simulink model "SimplePropellerModel"  (R2025b)
settings: Solver=VariableStepAuto  StartTime=0.0  StopTime=20  RelTol=1e-3
undefined symbols (not defined in the file): km, kT, spinDir
libraries: simulink x1
settings Model: Creator=esmithzb  LastModifiedBy=David
settings DebuggingCC: UnderspecifiedInitializationDetection=Classic  MergeDetectMultiDrivingBlocksExec=none
settings ModelReferenceCC: PropagateSignalLabelsOutOfModel=off

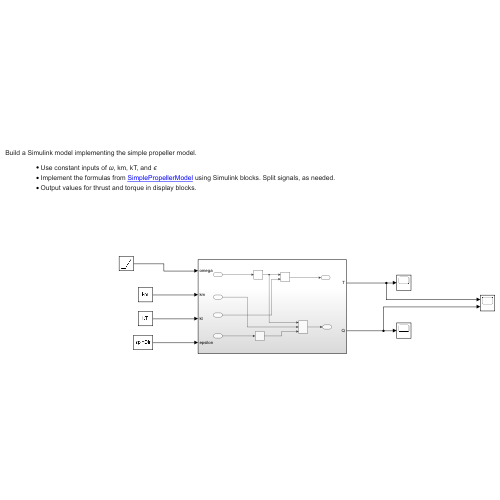
[thumbnail: Simulink's stored preview of the top-level diagram]
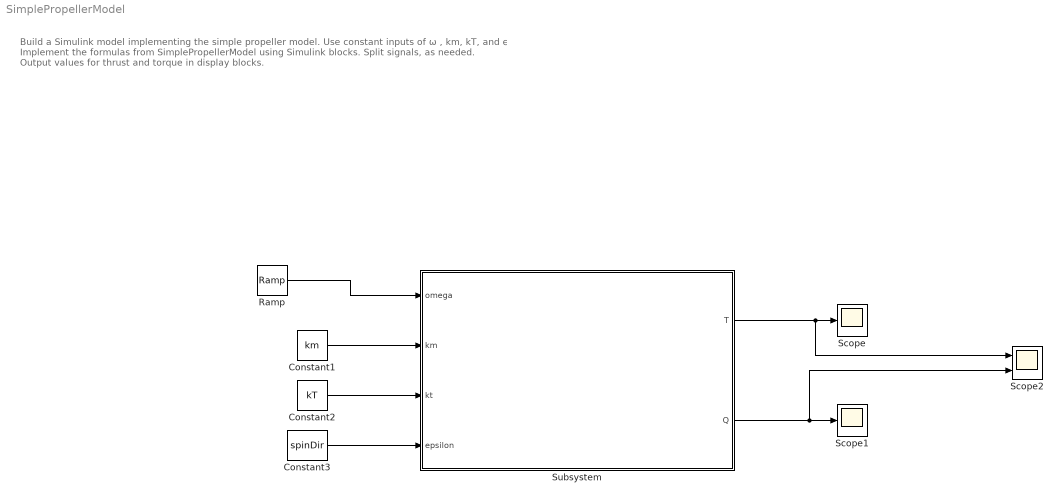
== system SimplePropellerModel ==
  note: Build a Simulink model implementing the simple propeller model.
      | Use constant inputs of ω , km, kT, and ϵ
      | Implement the formulas from SimplePropellerModel using Simulink blocks. Split signals, as needed.
      | Output values for thrust and torque in display blocks.
  Constant1 : Constant  Value=km
  Constant2 : Constant  Value=kT
  Constant3 : Constant  Value=spinDir
  Ramp : simulink/Sources/Ramp  slope=4.5  start=0  InitialOutput=0
  Scope : Scope
      settings: ActiveDisplayYMinimum=-0.018224999999999998  ActiveDisplayYMaximum=0.164025
  Scope1 : Scope
      settings: ActiveDisplayYMinimum=-0.00020249999999999993  ActiveDisplayYMaximum=0.0018225
  Scope2 : Scope  NumInputPorts=2
      settings: ActiveDisplayYMinimum=-0.018224999999999998  ActiveDisplayYMaximum=0.164025  DataLoggingVariableName=ScopeData2
  Subsystem : Subsystem
  wires:
  Ramp/1 -> Subsystem/1(omega)
  Constant3/1 -> Subsystem/4(epsilon)
  Constant2/1 -> Subsystem/3(kt)
  Constant1/1 -> Subsystem/2(km)
  Subsystem/1(T) -> Scope2/1, Scope/1
  Subsystem/2(Q) -> Scope2/2, Scope1/1

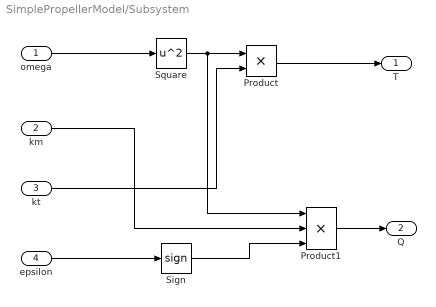
== system SimplePropellerModel/Subsystem ==
  omega : Inport
  km : Inport  Port=2
  kt : Inport  Port=3
  epsilon : Inport  Port=4
  Product : Product
  Product1 : Product  Inputs=3
  Sign : Signum
  Square : Math  Operator=square
  T : Outport
  Q : Outport  Port=2
  wires:
  omega/1 -> Square/1
  Square/1 -> Product1/1, Product/1
  Product/1 -> T/1
  kt/1 -> Product/2
  epsilon/1 -> Sign/1
  Product1/1 -> Q/1
  Sign/1 -> Product1/3
  km/1 -> Product1/2
